simulink model "case_14_state_oscillation"  (R2025b)
settings: Solver=VariableStepAuto  StartTime=0.0  StopTime=240  RelTol=1e-3
settings Model: Creator=sanborkl  LastModifiedBy=sanborkl

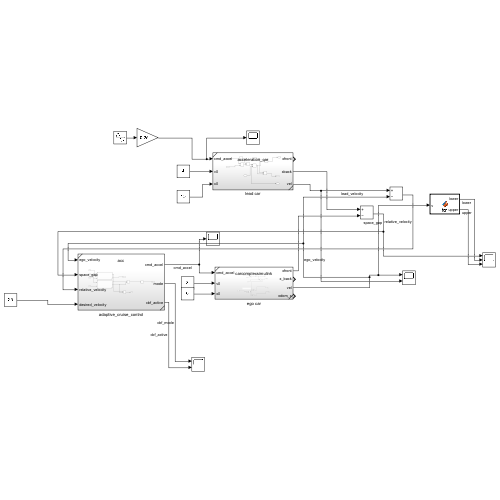
[thumbnail: Simulink's stored preview of the top-level diagram]
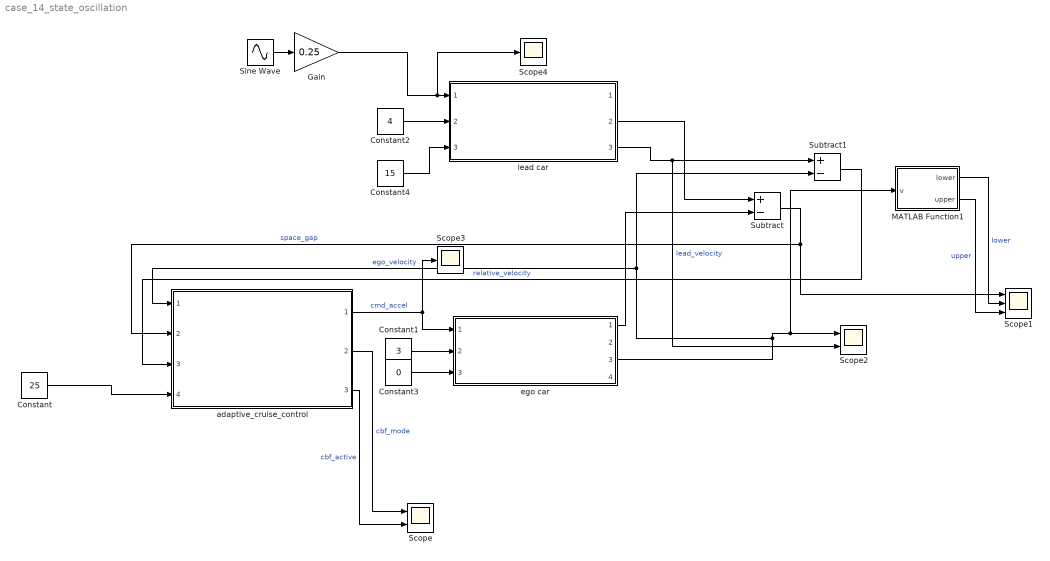
== system case_14_state_oscillation ==
  Constant : Constant  Value=25
  Constant1 : Constant  Value=3
  Constant2 : Constant  Value=4
  Constant3 : Constant  Value=0
  Constant4 : Constant  Value=15
  Gain : Gain  Gain=0.25
  MATLAB Function1 : MATLAB Function  TreatAsAtomicUnit=on
  Scope : Scope  NumInputPorts=2
      settings: ActiveDisplayYMinimum=0.75000000000000011  ActiveDisplayYMaximum=3.25
  Scope1 : Scope  NumInputPorts=3
      settings: ActiveDisplayYMinimum=8.2608936855825874  ActiveDisplayYMaximum=33.2519568297567  YLabel=m
  Scope2 : Scope  NumInputPorts=2
      settings: ActiveDisplayYMinimum=2.1252451140353159  ActiveDisplayYMaximum=10.872793973682157  YLabel=m/s  DataLoggingVariableName=ScopeData2
  Scope3 : Scope
      settings: ActiveDisplayYMinimum=-0.74079852174013494  ActiveDisplayYMaximum=1.7489776135266817  YLabel=m/s^2  DataLoggingVariableName=ScopeData3
  Scope4 : Scope
      settings: ActiveDisplayYMinimum=-0.31249932123657259  ActiveDisplayYMaximum=0.31249816376782075  DataLoggingVariableName=ScopeData4
  Sine Wave : Sin  Frequency=0.125  SampleTime=0
  Subtract : Sum  Inputs=+-
  Subtract1 : Sum  Inputs=+-
  adaptive_cruise_control : Subsystem  ReferencedSubsystem=acc
  ego car : Subsystem  ReferencedSubsystem=carcomplexsimulink
  lead car : Subsystem  ReferencedSubsystem=acceleration_car
  wires:
  ego car/3 -> Scope2/1, MATLAB Function1/1(v), Subtract1/2, adaptive_cruise_control/1  "ego_velocity"
  adaptive_cruise_control/1 -> ego car/1, Scope3/1  "cmd_accel"
  Constant1/1 -> ego car/2
  Subtract1/1 -> adaptive_cruise_control/3  "relative_velocity"
  lead car/3 -> Scope2/2, Subtract1/1  "lead_velocity"
  Constant3/1 -> ego car/3
  Sine Wave/1 -> Gain/1
  Constant2/1 -> lead car/2
  adaptive_cruise_control/2 -> Scope/1  "cbf_mode"
  lead car/2 -> Subtract/1
  adaptive_cruise_control/3 -> Scope/2  "cbf_active"
  Constant/1 -> adaptive_cruise_control/4
  ego car/1 -> Subtract/2
  Subtract/1 -> Scope1/1, adaptive_cruise_control/2  "space_gap"
  Constant4/1 -> lead car/3
  Gain/1 -> Scope4/1, lead car/1
  MATLAB Function1/1(lower) -> Scope1/2  "lower"
  MATLAB Function1/2(upper) -> Scope1/3  "upper"

== matlab function case_14_state_oscillation/MATLAB Function1 ==
  data: v input; lower output; upper output
function [lower, upper] = fcn(v)

lower = 2 * v + 5;
upper = 2 * v + 15;
